simulink model "simscape"  (R2020b)
settings: Solver=VariableStepAuto  StartTime=0.0  StopTime=10  FixedStep=0.0001  MaxStep=0.1  RelTol=1e-3  EnableMultiTasking=on
model workspace (MAT data in the model file):
  m_ges = Simulink.Parameter
  m_ges.DataType = 'auto'
  m_ges.Dimensions = [0 0]
values from neighbouring files (symbols this model uses):
  c = 10    [simscape_variables.m]
  c_phi = 0.4    [simscape_variables.m]
  F1 = 2    [simscape_variables.m]
  g = 9.80665    [simscape_variables.m]
  gain_4 = 1/(l_1^2*(m_1/3 + m_3))    (= 187.5)    [simscape_variables.m]
  k = 10    [simscape_variables.m]
  k_phi = 40    [simscape_variables.m]
  l_1 = 0.2    [simscape_variables.m]
  M1 = 30    [simscape_variables.m]
  m_1 = 0.1    [simscape_variables.m]
  m_2 = 0.1    [simscape_variables.m]
  m_3 = 0.1    [simscape_variables.m]
  m_s = m_1/2 + m_3    (= 0.15)    [simscape_variables.m]
  omega_0 = 10    [simscape_variables.m]
undefined symbols (not defined in the file or in its folder): X, Y, Z
libraries: sm_lib x12, nesl_utility x5
settings Model: Creator=The MathWorks, Inc.
settings DataIOCC: LimitDataPoints=on  SaveFormat=Array  ReturnWorkspaceOutputs=off
settings OptimizationCC: LifeSpan=inf
settings DebuggingCC: UnderspecifiedInitializationDetection=Classic  MergeDetectMultiDrivingBlocksExec=none  SolverPrmCheckMsg=warning  SFUnexpectedBacktrackingDiag=warning  SFNoUnconditionalDefaultTransitionDiag=warning  SFExecutionAtInitializationDiag=none  ArithmeticOperatorsInVariantConditions=warning
settings HardwareCC: ProdBitPerPointer=32  ProdBitPerSizeT=32  ProdBitPerPtrDiffT=32  ProdLargestAtomicFloat=None  ProdIntDivRoundTo=Undefined  ProdEndianess=Unspecified  ProdWordSize=32  ProdHWDeviceType=32-bit Generic
settings ModelReferenceCC: PropagateSignalLabelsOutOfModel=off
settings SFSimCC: SimUseLocalCustomCode=off  CustomCodeUndefinedFunction=UseInterfaceOnly
settings RTWCC: RTWUseLocalCustomCode=off
settings CodeAppCC: StateflowObjectComments=on
settings GRTTargetCC: TargetLangStandard=C89/C90 (ANSI)
settings ConfigComp: CovMetricSettings=dw  CovSaveCumulativeToWorkspaceVar=on  CovSaveSingleToWorkspaceVar=on  CovExternalEMLEnable=off
settings SimscapeCC: SimscapeNormalizeSystem=off
settings ConfigurationSet: Description=SimMechanics 2G
settings DiagnosticsConfigSet: SimMechanicsUnconnectedFramePorts=none
settings ExplorerConfigSet: InternalSimMechanicsExplorerSettings="<ExplorerConfiguration><canonicalview>default</canonicalview><TilePanel><TileInfo><Tiles Columns=\"1\" Count=\"1\" Rows=\"1\"><Column Left=\"2\" Weight=\"1\"/><Column Left=\"533\"/><Row Top=\"2\" Weight=\"1\"/><Row Top=\"371\"/><Tile Height=\"1\" Width=\"1\" X=\"0\" Y=\"0\"/></Tiles></TileInfo><SceneInfo><SceneViewer><BGColor><R>0.80000001192092896</R><G>0.80000001192092896</G><B>0.80000001192092896</B></BGColor><Camera><Position><X>0.43420936018603001</X><Y>-0.4103794555707736</Y><Z>0.11459195051504517</Z></Position><Center><X>0.032157478757701863</X><Y>-0.008327574142445426</Y><Z>-0.28745993091328081</Z></Center><Up><X>-0.40824829046386307</X><Y>0.40824829046386307</Y><Z>0.81649658092772615</Z></Up><Left>-0.11196334282447423</Left><Right>0.11196334282447423</Right><Bottom>-0.30046102603105562</Bottom><Top>0.30046102603105562</Top></Camera></SceneViewer></SceneInfo></TilePanel></ExplorerConfiguration>"

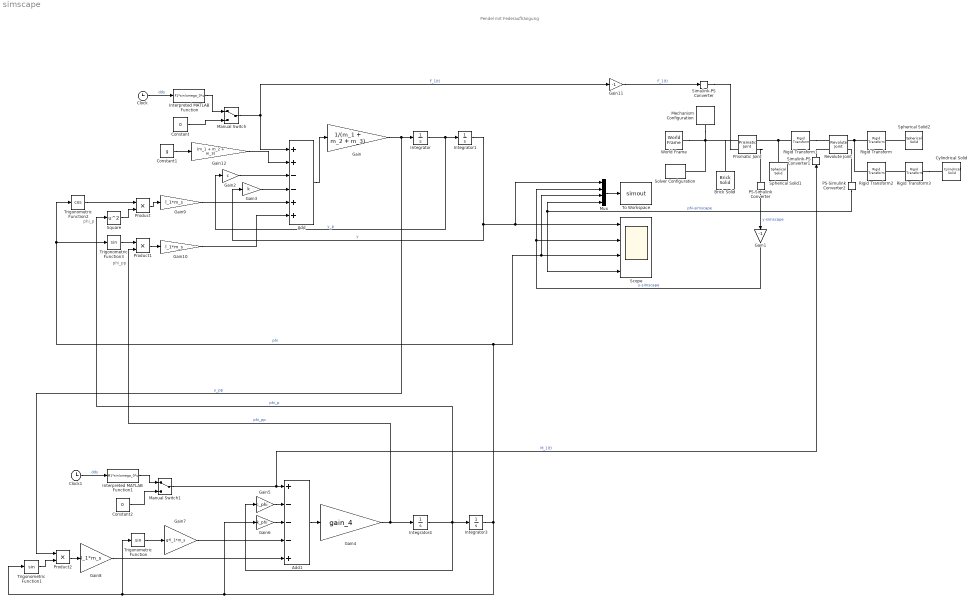
== system simscape ==
  note: phi_pp
  note: phi_p
  note: Pendel mit Federaufhängung
  Add : Sum  Inputs=++--++
  Add1 : Sum  Inputs=+---+
  Brick Solid : sm_lib/Body Elements/Brick Solid  GraphicAmbientColor=[0.15 0.15 0.15 1.0]  BasedOnType=Density  BrickDimensions=[0.1 0.1 0.01]  BrickDimensionUnits=m  CenterOfMass=[0 0 0]  CenterOfMassUnits=m  GraphicDiffuseColor=[0.5 0.5 0.5]  Density=1000  DensityUnits=kg/m^3  DoExposeReferenceFrame=on  GraphicEmissiveColor=[0.0 0.0 0.0 1.0]  ExportEntireGeometry=off  SerializedFrames=<Frames/>  MarkerShape=Sphere  MarkerSize=10  GraphicType=FromGeometry  InertiaType=CalculateFromGeometry  Mass=1  MassUnits=kg  MomentsOfInertia=[1 1 1]  MomentsOfInertiaUnits=kg*m^2  GraphicOpacity=1.0  ProductsOfInertia=[0 0 0]  ProductsOfInertiaUnits=kg*m^2  GraphicShininess=75  GraphicSpecularColor=[0.5 0.5 0.5 1.0]  GraphicVisPropType=SimpleVisualProperties
  Clock : Clock
  Clock1 : Clock
  Constant : Constant  Value=0
  Constant1 : Constant  Value=g
  Constant2 : Constant  Value=0
  Cylindrical Solid : sm_lib/Body Elements/Cylindrical Solid  GraphicAmbientColor=[0.15 0.15 0.15 1.0]  BasedOnType=Mass  CenterOfMass=[0 0 0]  CenterOfMassUnits=m  GraphicDiffuseColor=[1.0 0.2 0.4]  CylinderLength=l_1  CylinderLengthUnits=m  CylinderRadius=0.005  CylinderRadiusUnits=m  Density=1000  DensityUnits=kg/m^3  DoExposeReferenceFrame=on  GraphicEmissiveColor=[0.0 0.0 0.0 1.0]  ExportEntireGeometry=off  SerializedFrames=<Frames/>  MarkerShape=Sphere  MarkerSize=10  GraphicType=FromGeometry  InertiaType=CalculateFromGeometry  Mass=m_1  MassUnits=kg  MomentsOfInertia=[1 1 1]  MomentsOfInertiaUnits=kg*m^2  GraphicOpacity=0.3  ProductsOfInertia=[0 0 0]  ProductsOfInertiaUnits=kg*m^2  GraphicShininess=75  GraphicSpecularColor=[0.5 0.5 0.5 1.0]  GraphicVisPropType=SimpleVisualProperties
  Gain : Gain  Gain=1/(m_1 + m_2 + m_3)
  Gain1 : Gain  Gain=-1
  Gain10 : Gain  Gain=l_1*m_s
  Gain11 : Gain  Gain=-1
  Gain12 : Gain  Gain=(m_1 + m_2 + m_3)
  Gain2 : Gain  Gain=c
  Gain3 : Gain  Gain=k
  Gain4 : Gain  Gain=gain_4
  Gain5 : Gain  Gain=c_phi
  Gain6 : Gain  Gain=k_phi
  Gain7 : Gain  Gain=g*l_1*m_s
  Gain8 : Gain  Gain=l_1*m_s
  Gain9 : Gain  Gain=l_1*m_s
  Integrator{,1,3..4} (4 alike) : Integrator
  Interpreted MATLAB Function : MATLABFcn  MATLABFcn=F1*sin(omega_0*u)
  Interpreted MATLAB Function1 : MATLABFcn  MATLABFcn=M1*sin(omega_0*u)
  Manual Switch : ManualSwitch
  Manual Switch1 : ManualSwitch
  Mechanism Configuration : sm_lib/Utilities/Mechanism Configuration  UniformGravity=Constant  GravityVector=[0 0 -9.80665]  GravityVectorUnits=m/s^2  GravityUnits=m/s^2  LinearizationDelta=0.001  JointModeTransitionNonlinearIterations=2
      settings: SourceProductName=Multibody
  Mux : Mux
  PS-Simulink Converter : nesl_utility/PS-Simulink Converter  PhysicalDomain=network_engine_domain  SubClassName=ps_output  LeftPortType=input  RightPortType=output  PseudoPeriodic=off  Frequencies=[]  Unit=inherit  AffineConversion=off
  PS-Simulink Converter2 : nesl_utility/PS-Simulink Converter  PhysicalDomain=network_engine_domain  SubClassName=ps_output  LeftPortType=input  RightPortType=output  PseudoPeriodic=off  Frequencies=[]  Unit=inherit  AffineConversion=off
  Prismatic Joint : sm_lib/Joints/Prismatic Joint  JointMode=Normal  SenseConstraintForce=off  SenseConstraintForceX=off  SenseConstraintForceY=off  SenseConstraintForceZ=off  SenseConstraintTorque=off  SenseConstraintTorqueX=off  SenseConstraintTorqueY=off  SenseConstraintTorqueZ=off  SenseTotalForce=off  SenseTotalForceX=off  SenseTotalForceY=off  SenseTotalForceZ=off  SenseTotalTorque=off  SenseTotalTorqueX=off  SenseTotalTorqueY=off  SenseTotalTorqueZ=off  CompositeWrenchDir=FollowerOnBase  CompositeWrenchFrame=BaseFrame  EquilibriumPosition=0  EquilibriumPositionUnits=m  SpringStiffness=k  SpringStiffnessUnits=N/m  DampingCoefficient=c  DampingCoefficientUnits=N/(m/s)  TorqueActuationMode=InputTorque  MotionActuationMode=ComputedMotion  SensePosition=on  SenseVelocity=off  SenseAcceleration=off  SenseTorqueForce=off  SenseLowerLimitTorqueForce=off  SenseUpperLimitTorqueForce=off  LowerLimitSpecify=off  LowerLimitBound=-1  LowerLimitBoundUnits=m  LowerLimitStiffness=1e6  LowerLimitStiffnessUnits=N/m  LowerLimitDamping=1e3  LowerLimitDampingUnits=N/(m/s)  LowerLimitTransitionRegionWidth=1e-4  LowerLimitTransitionRegionWidthUnits=m  UpperLimitSpecify=off  UpperLimitBound=1  UpperLimitBoundUnits=m  UpperLimitStiffness=1e6  UpperLimitStiffnessUnits=N/m  UpperLimitDamping=1e3  UpperLimitDampingUnits=N/(m/s)  UpperLimitTransitionRegionWidth=1e-4  UpperLimitTransitionRegionWidthUnits=m  PositionTargetSpecify=on  PositionTargetPriority=High  PositionTargetValue=0  PositionTargetValueUnits=m  VelocityTargetSpecify=on  VelocityTargetPriority=High  VelocityTargetValue=0  VelocityTargetValueUnits=m/s
  Product : Product
  Product1 : Product
  Product2 : Product
  Revolute Joint : sm_lib/Joints/Revolute Joint  JointMode=Normal  SenseConstraintForce=off  SenseConstraintForceX=off  SenseConstraintForceY=off  SenseConstraintForceZ=off  SenseConstraintTorque=off  SenseConstraintTorqueX=off  SenseConstraintTorqueY=off  SenseConstraintTorqueZ=off  SenseTotalForce=off  SenseTotalForceX=off  SenseTotalForceY=off  SenseTotalForceZ=off  SenseTotalTorque=off  SenseTotalTorqueX=off  SenseTotalTorqueY=off  SenseTotalTorqueZ=off  CompositeWrenchDir=FollowerOnBase  CompositeWrenchFrame=BaseFrame  EquilibriumPosition=0  EquilibriumPositionUnits=rad  SpringStiffness=k_phi  SpringStiffnessUnits=N*m/rad  DampingCoefficient=c_phi  DampingCoefficientUnits=N*m/(rad/s)  TorqueActuationMode=InputTorque  MotionActuationMode=ComputedMotion  SensePosition=on  SenseVelocity=off  SenseAcceleration=off  SenseTorqueForce=off  SenseLowerLimitTorqueForce=off  SenseUpperLimitTorqueForce=off  LowerLimitSpecify=off  LowerLimitBound=-90  LowerLimitBoundUnits=deg  LowerLimitStiffness=1e4  LowerLimitStiffnessUnits=N*m/deg  LowerLimitDamping=10  LowerLimitDampingUnits=N*m/(deg/s)  LowerLimitTransitionRegionWidth=0.1  LowerLimitTransitionRegionWidthUnits=deg  UpperLimitSpecify=off  UpperLimitBound=90  UpperLimitBoundUnits=deg  UpperLimitStiffness=1e4  UpperLimitStiffnessUnits=N*m/deg  UpperLimitDamping=10  UpperLimitDampingUnits=N*m/(deg/s)  UpperLimitTransitionRegionWidth=0.1  UpperLimitTransitionRegionWidthUnits=deg  PositionTargetSpecify=on  PositionTargetPriority=High  PositionTargetValue=0  PositionTargetValueUnits=rad  VelocityTargetSpecify=on  VelocityTargetPriority=High  VelocityTargetValue=0  VelocityTargetValueUnits=rad/s
      settings: SourceProductName=Multibody
  Rigid Transform : sm_lib/Frames and Transforms/Rigid Transform  TranslationMethod=StandardAxis  TranslationStandardOffset=-l_1  TranslationLengthUnit=m  TranslationStandardAxis=+Y  TranslationCartesianOffset=[0 0 0]  TranslationROffset=0  TranslationROffsetUnits=m  TranslationZOffset=0  TranslationZOffsetUnits=m  TranslationThetaOffset=0  TranslationThetaOffsetUnits=deg  RotationMethod=None  RotationAngleUnits=deg  RotationStandardAxis=-Z  RotationAngle=10  RotationArbitraryAxis=[0 0 1]  FollAlignAxisA=+X  BaseAlignAxisA=+Y  FollAlignAxisB=+Y  BaseAlignAxisB=+Z  RotationSequenceAxes=FollowerAxes  RotationSequence=XYX  RotationSequenceAngles=[0 0 0]  RotationSequenceAnglesUnits=deg  RotationMatrix=[1 0 0; 0 1 0; 0 0 1]
  Rigid Transform1 : sm_lib/Frames and Transforms/Rigid Transform  TranslationMethod=None  TranslationStandardOffset=0  TranslationLengthUnit=m  TranslationStandardAxis=+Z  TranslationCartesianOffset=[0 0 0]  TranslationROffset=0  TranslationROffsetUnits=m  TranslationZOffset=0  TranslationZOffsetUnits=m  TranslationThetaOffset=0  TranslationThetaOffsetUnits=deg  RotationMethod=StandardAxis  RotationAngleUnits=deg  RotationStandardAxis=+X  RotationAngle=90  RotationArbitraryAxis=[0 0 1]  FollAlignAxisA=+X  BaseAlignAxisA=+Y  FollAlignAxisB=+Y  BaseAlignAxisB=+Z  RotationSequenceAxes=FollowerAxes  RotationSequence=XYX  RotationSequenceAngles=[0 0 0]  RotationSequenceAnglesUnits=deg  RotationMatrix=[1 0 0; 0 1 0; 0 0 1]
  Rigid Transform2 : sm_lib/Frames and Transforms/Rigid Transform  TranslationMethod=None  TranslationStandardOffset=0  TranslationLengthUnit=m  TranslationStandardAxis=+Z  TranslationCartesianOffset=[0 0 0]  TranslationROffset=0  TranslationROffsetUnits=m  TranslationZOffset=0  TranslationZOffsetUnits=m  TranslationThetaOffset=0  TranslationThetaOffsetUnits=deg  RotationMethod=StandardAxis  RotationAngleUnits=deg  RotationStandardAxis=+X  RotationAngle=90  RotationArbitraryAxis=[0 0 1]  FollAlignAxisA=+X  BaseAlignAxisA=+Y  FollAlignAxisB=+Y  BaseAlignAxisB=+Z  RotationSequenceAxes=FollowerAxes  RotationSequence=XYX  RotationSequenceAngles=[0 0 0]  RotationSequenceAnglesUnits=deg  RotationMatrix=[1 0 0; 0 1 0; 0 0 1]
  Rigid Transform3 : sm_lib/Frames and Transforms/Rigid Transform  TranslationMethod=StandardAxis  TranslationStandardOffset=l_1/2  TranslationLengthUnit=m  TranslationStandardAxis=+Z  TranslationCartesianOffset=[0 0 0]  TranslationROffset=0  TranslationROffsetUnits=m  TranslationZOffset=0  TranslationZOffsetUnits=m  TranslationThetaOffset=0  TranslationThetaOffsetUnits=deg  RotationMethod=None  RotationAngleUnits=deg  RotationStandardAxis=-Z  RotationAngle=10  RotationArbitraryAxis=[0 0 1]  FollAlignAxisA=+X  BaseAlignAxisA=+Y  FollAlignAxisB=+Y  BaseAlignAxisB=+Z  RotationSequenceAxes=FollowerAxes  RotationSequence=XYX  RotationSequenceAngles=[0 0 0]  RotationSequenceAnglesUnits=deg  RotationMatrix=[1 0 0; 0 1 0; 0 0 1]
  Scope : Scope  NumInputPorts=4
  Simulink-PS Converter : nesl_utility/Simulink-PS Converter  PhysicalDomain=network_engine_domain  SubClassName=ps_input  LeftPortType=input  RightPortType=output  PseudoPeriodic=off  Frequencies=[]  NoiseDistribution=none  NoiseParameters=[]  Unit=1  AffineConversion=off  FilteringAndDerivatives=provide  SimscapeFilterOrder=1  InputFilterTimeConstant=0.001  UdotUserProvided=0
  Simulink-PS Converter1 : nesl_utility/Simulink-PS Converter  PhysicalDomain=network_engine_domain  SubClassName=ps_input  LeftPortType=input  RightPortType=output  PseudoPeriodic=off  Frequencies=[]  NoiseDistribution=none  NoiseParameters=[]  Unit=1  AffineConversion=off  FilteringAndDerivatives=provide  SimscapeFilterOrder=1  InputFilterTimeConstant=0.001  UdotUserProvided=0
  Solver Configuration : nesl_utility/Solver Configuration  PhysicalDomain=network_engine_domain  SubClassName=solver  LeftPortType=input  RightPortType=generic  Tones=[]  Harmonics=[]  SimulateNoise=off  Profile=off  UseLocalSampling=off  EnableSwitchedLinearOptims=on  FrequencyDomain=off  UseCCode=off  RelTol=0.001  AbsTol=1e-06  MinStep=1e-09  ToWorkspace=off  RevertToSquareIcSolve=off  NumHomotopyIterations=100  PhasorMode=off  PhasorModeNumHarmonics=1  DoDC=off  ResidualTolerance=1e-03  UseLocalSolver=off  LocalSolverChoice=NE_BACKWARD_EULER_ADVANCER  LocalSolverSampleTime=0.001  DoFixedCost=off  MaxNonlinIter=3  MaxModeIter=2  ComputeImpulses=off  ImpulseIterations=2  LinearAlgebra=Sparse  EquationFormulation=NE_TIME_EF  DelaysMemoryBudget=1024  AutomaticFiltering=on  FilteringTimeConstant=0.001  PartitionStorageMethod=AS_NEEDED  PartitionMemoryBudget=1024  PartitionMethod=FAST
      settings: SourceProductName=Utilities
  Spherical Solid1 : sm_lib/Body Elements/Spherical Solid  GraphicAmbientColor=[0.15 0.15 0.15 1.0]  BasedOnType=Mass  CenterOfMass=[0 0 0]  CenterOfMassUnits=m  GraphicDiffuseColor=[0.5 0.5 0.5]  Density=1000  DensityUnits=kg/m^3  DoExposeReferenceFrame=on  GraphicEmissiveColor=[0.0 0.0 0.0 1.0]  ExportEntireGeometry=off  SerializedExposedGeometries=<ExposedGeometries/>  SerializedFrames=<Frames/>  MarkerShape=Sphere  MarkerSize=10  GraphicType=FromGeometry  InertiaType=CalculateFromGeometry  Mass=m_2  MassUnits=kg  MomentsOfInertia=[1 1 1]  MomentsOfInertiaUnits=kg*m^2  GraphicOpacity=1.0  ProductsOfInertia=[0 0 0]  ProductsOfInertiaUnits=kg*m^2  GraphicShininess=75  GraphicSpecularColor=[0.5 0.5 0.5 1.0]  SphereRadius=0.01  SphereRadiusUnits=m  GraphicVisPropType=SimpleVisualProperties
  Spherical Solid2 : sm_lib/Body Elements/Spherical Solid  GraphicAmbientColor=[0.15 0.15 0.15 1.0]  BasedOnType=Mass  CenterOfMass=[0 0 0]  CenterOfMassUnits=m  GraphicDiffuseColor=[0.5 0.5 0.5]  Density=10000  DensityUnits=kg/m^3  DoExposeReferenceFrame=on  GraphicEmissiveColor=[0.0 0.0 0.0 1.0]  ExportEntireGeometry=off  SerializedExposedGeometries=<ExposedGeometries/>  SerializedFrames=<Frames/>  MarkerShape=Sphere  MarkerSize=10  GraphicType=FromGeometry  InertiaType=CalculateFromGeometry  Mass=m_3  MassUnits=kg  MomentsOfInertia=[1 1 1]  MomentsOfInertiaUnits=kg*m^2  GraphicOpacity=1.0  ProductsOfInertia=[0 0 0]  ProductsOfInertiaUnits=kg*m^2  GraphicShininess=75  GraphicSpecularColor=[0.5 0.5 0.5 1.0]  SphereRadius=0.01  SphereRadiusUnits=m  GraphicVisPropType=SimpleVisualProperties
  Square : Math  Operator=square  SaturateOnIntegerOverflow=on
  To Workspace : ToWorkspace  VariableName=simout  SampleTime=-1
      settings: Save2DSignal=2-D array (concatenate along first dimension)
  Trigonometric Function : Trigonometry
  Trigonometric Function1 : Trigonometry
  Trigonometric Function2 : Trigonometry  Operator=cos
  Trigonometric Function3 : Trigonometry
  World Frame : sm_lib/Frames and Transforms/World Frame
      settings: SourceProductName=Multibody
  wires:
  Clock/1 -> Interpreted MATLAB Function/1  "dds"
  Interpreted MATLAB Function/1 -> Manual Switch/1
  Constant/1 -> Manual Switch/2
  Manual Switch/1 -> Add/1, Gain11/1  "F_1(t)"
  Add/1 -> Gain/1
  Gain12/1 -> Add/2
  Constant1/1 -> Gain12/1
  Gain/1 -> Product2/1, Integrator/1  "y_pp"
  Integrator/1 -> Integrator1/1, Gain2/1  "y_p"
  Gain2/1 -> Add/3
  Gain3/1 -> Add/4
  Integrator1/1 -> Mux/1, Scope/1, Gain3/1  "y"
  Add1/1 -> Gain4/1
  Interpreted MATLAB Function1/1 -> Manual Switch1/1
  Constant2/1 -> Manual Switch1/2
  Clock1/1 -> Interpreted MATLAB Function1/1  "dds"
  Manual Switch1/1 -> Simulink-PS Converter1/1, Add1/1  "M_1(t)"
  Gain4/1 -> Product1/2, Integrator4/1  "phi_pp"
  Integrator4/1 -> Gain5/1, Integrator3/1, Square/1  "phi_p"
  Trigonometric Function/1 -> Gain7/1
  Trigonometric Function1/1 -> Product2/2
  Product2/1 -> Gain8/1
  Square/1 -> Product/2
  Trigonometric Function3/1 -> Product1/1
  Product1/1 -> Gain10/1
  Product/1 -> Gain9/1
  Trigonometric Function2/1 -> Product/1
  Integrator3/1 -> Trigonometric Function/1, Trigonometric Function1/1, Gain6/1, Trigonometric Function3/1, Trigonometric Function2/1, Mux/3, Scope/3  "phi"
  Gain5/1 -> Add1/2
  Gain6/1 -> Add1/3
  Gain8/1 -> Add1/5
  PS-Simulink Converter2/1 -> Scope/4, Mux/4  "phi-simscape"
  Gain7/1 -> Add1/4
  Gain10/1 -> Add/6
  Gain9/1 -> Add/5
  Gain11/1 -> Simulink-PS Converter/1  "F_1(t)"
  PS-Simulink Converter/1 -> Gain1/1  "y-simscape"
  Gain1/1 -> Mux/2, Scope/2  "y-simscape"
  Mux/1 -> To Workspace/1
  connections:
  Mechanism Configuration/RConn1 -- Solver Configuration/RConn1 -- World Frame/RConn1 -- Prismatic Joint/LConn1 -- Brick Solid/RConn1
  Rigid Transform/LConn1 -- Rigid Transform2/LConn1 -- Revolute Joint/RConn1
  Spherical Solid2/RConn1 -- Rigid Transform/RConn1
  Spherical Solid1/RConn1 -- Prismatic Joint/RConn1 -- Rigid Transform1/LConn1
  Rigid Transform1/RConn1 -- Revolute Joint/LConn1
  Simulink-PS Converter/RConn1 -- Prismatic Joint/LConn2
  Revolute Joint/LConn2 -- Simulink-PS Converter1/RConn1
  Rigid Transform3/LConn1 -- Rigid Transform2/RConn1
  Rigid Transform3/RConn1 -- Cylindrical Solid/RConn1
  Prismatic Joint/RConn2 -- PS-Simulink Converter/LConn1
  PS-Simulink Converter2/LConn1 -- Revolute Joint/RConn2
